simulink model "TractorTransmissionTradeOff"  (R2025a)
settings: Solver=daessc  StartTime=0.0  StopTime=125  RelTol=1e-3  AbsTol=1e-3
PreLoadFcn:
  | distanceVector = [0,0.1389,0.4167,0.8333,1.3889,2.0833,2.9167,3.889,5,6.25,7.6389,200];
  | targetVelocityVector = [0,0.5,1,1.5,2,2.5,3,3.5,4,4.5,5,5];
InitFcn:
  | TractorEnergyComputationInput
undefined symbols (not defined in the file or in its folder): engine, implement, tc, tire, tk, tphi, tykc, tykphi, tyn
libraries: nesl_utility x33, fl_lib x18, sdl_lib x6, simulink x5, slpidlib x1
(part 1 of 3)
CloseFcn:
  | try,close(hTractorTransmissionTradeOff),end
  | clear hTractorTransmissionTradeOff
  | 
  | clear tout simlogTractorTransmissionTradeOff
  | clear logsoutTractorTransmissionTradeOff
  | 
  | clear driveline engine finalDrive
  | clear hydrostaticCVT pump tire implement
  | clear h1_plotEnergySankey
Description:
  | Tractor Transmission Energy Flow Chart
settings Model: Creator=The MathWorks, Inc.  LastModifiedBy=varora
settings SolverCC: AutoScaleAbsTol=off  MaxConsecutiveMinStep=10  AlgebraicLoopSolver=TrustRegion  MaxZcPerStep=1.0
settings DataIOCC: DSMLogging=off  ReturnWorkspaceOutputs=off  SignalLoggingName=logsoutTractorTransmissionTradeOff
settings OptimizationCC: ReuseModelBlockBuffer=off
settings DebuggingCC: IgnoredZcDiagnostic=none  UnconnectedInputMsg=warning  UnconnectedOutputMsg=warning  UnconnectedLineMsg=warning  SymbolicDimsDataTypeCodeGenerationDiagnostic=none
settings ModelReferenceCC: EnableRefExpFcnMdlSchedulingChecks=on
settings SFSimCC: CustomCodeUndefinedFunction=UseInterfaceOnly
settings RTWCC: GPUComputeCapability=3.5  DLArmComputeVersion=19.05
settings SimscapeCC: SimscapeLogName=simlogTractorTransmissionTradeOff  SimscapeLogDataHistory=1000000.0

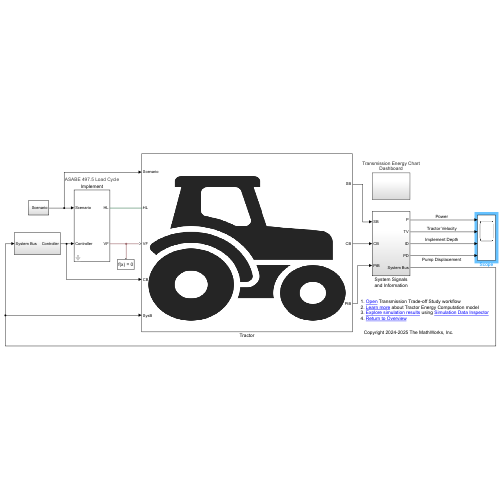
[thumbnail: Simulink's stored preview of the top-level diagram]
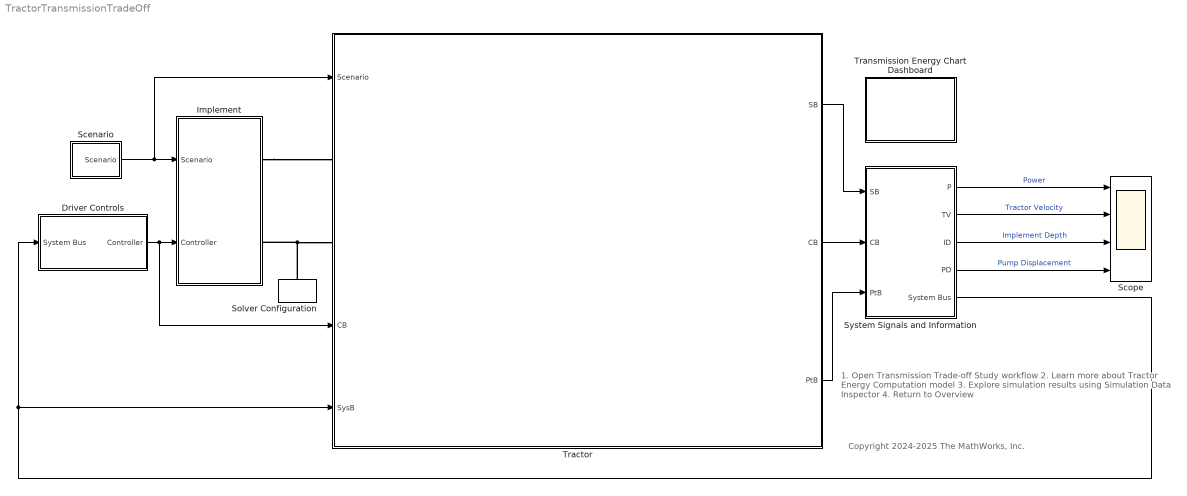
== system TractorTransmissionTradeOff ==
  note: Copyright 2024-2025 The MathWorks, Inc.
  note: 1. Open Transmission Trade-off Study workflow
      | 2. Learn more about Tractor Energy Computation model
      | 3. Explore simulation results using Simulation Data Inspector
      | 4. Return to Overview
  Driver Controls : Subsystem
  Implement : Subsystem  Tag=ASABE 497.5 Load Cycle  Description=ASABE 497.5 Load Cycle  mask{methodForceComputation=Draft force prediction based on ASABE D497.5 standard, typeImplement=Chisel Plow - 5 cm straight point, widthImplement=1, numberTools=implement.numberTools, angleRake=implement.angleRake, vectorVelocity=[-1,0,0.05,0.5,1,1.5], vectorDraft=[-2.5,0,1800,2260,2480,2700], vectorVF=[0.5,0,-480,-525,-580,-620]}
      mask prompts: methodForceComputation "Draft (horizontal) force and vertical force computation"; typeImplement "Implement type"; widthImplement "Implement width (m)"; numberTools "Number of tools"; angleRake "Implement rake angle (deg)"; vectorVelocity "Velocity vector (m/s)"; vectorDraft "Draft force vector (N)"; vectorVF "Vertical force vector (N)"
      settings: AttributesFormatString=%<Tag>
      mask Callback methodForceComputation: ImplementMask
      mask Callback typeImplement: ImplementMask
      mask Callback widthImplement: ImplementMask
      mask Callback numberTools: ImplementMask
      mask Callback angleRake: ImplementMask
      mask Callback vectorVelocity: ImplementMask
      mask Callback vectorDraft: ImplementMask
      mask Callback vectorVF: ImplementMask
  Scenario : Subsystem
      settings: PortSchema="{\"entries\":[{\"content\":{\"sides\":[{\"content\":{\"connectorIds\":[\"Out1\"]},\"type\":\"ConnectorPlacement.EquallySpacedRectSide\",\"uuid\":\"b29e7b9e-789a-4413-ae11-5995fbedc15e\"},{\"content\":{\"side\":\"RIGHT\"},\"type\":\"ConnectorPlacement.EquallySpacedRectSide\",\"uuid\":\"46779515-8d36-4954-9a1a-0bbe9b69e0ab\"},{\"content\":{\"side\":\"TOP\"},\"type\":\"ConnectorPlacement.EquallySpacedRectSide\",\"uuid\":\"af37b6bf-e8aa-4a9f-b639-d899b0359ee5\"}]},\"type\":\"ConnectorPlacement.EquallySpacedConnector\",\"uuid\":\"f01fcd35-a429-4c8a-8cd6-eccdc9914f9f\"}],\"packageUris\":[\"http://schema.mathworks.com/mf0/Connector/R2020b\"],\"version\":\"1.0\"}"
  Scope : Scope  NumInputPorts=4
      settings: Title=Power, CVT (kW)  ActiveDisplayYMinimum=-3.21446  ActiveDisplayYMaximum=28.93014
  Solver Configuration : nesl_utility/Solver Configuration  PhysicalDomain=network_engine_domain  SubClassName=solver  LeftPortType=input  RightPortType=generic  Tones=[]  Harmonics=[]  SimulateNoise=off  Profile=off  UseLocalSampling=off  EnableSwitchedLinearOptims=on  FrequencyDomain=off  UseCCode=off  RelTol=0.001  AbsTol=1e-06  MinStep=1e-09  ToWorkspace=off  RevertToSquareIcSolve=off  NumHomotopyIterations=100  PhasorMode=off  PhasorModeNumHarmonics=1  ConsistencySolver=NEWTON_FTOL  IndexReductionMethod=DerivativeReplacement  DoDC=off  ResidualTolerance=1e-09  ConsistencyTolSource=GLOBAL  ConsistencyAbsTol=0.001  ConsistencyRelTol=0.001  ConsistencyTolFactor=0.001  UseLocalSolver=off  LocalSolverChoice=NE_BACKWARD_EULER_ADVANCER  ResolveIndetEquations=on  FunctionEvalNumThread=1  LocalSolverSampleTime=1e-5  DoFixedCost=off  MaxNonlinIter=6  MaxModeIter=2  ComputeImpulses=off  ImpulseIterations=2  LinearAlgebra=auto  LinearAlgebraNumThread=0  EquationFormulation=NE_TIME_EF  DelaysMemoryBudget=1024  AutomaticFiltering=on  FilteringTimeConstant=0.001  PartitionStorageMethod=AS_NEEDED  PartitionMemoryBudget=1024  PartitionMethod=ROBUST  MultibodyUseLocalSolver=off  MultibodyLocalSolverChoice=ODE1  MultibodyLocalSolverSampleTime=0.001
  System Signals and Information : Subsystem
  Tractor : Subsystem
      settings: PortSchema="{\"entries\":[{\"content\":{\"sides\":[{\"content\":{\"connectorIds\":[\"In1\",\"LConn1\",\"LConn2\",\"In2\",\"In3\"]},\"type\":\"ConnectorPlacement.EquallySpacedRectSide\",\"uuid\":\"54713dc4-af1f-4753-ac81-fb7b321017cb\"},{\"content\":{\"connectorIds\":[\"Out1\",\"Out2\",\"Out3\"],\"side\":\"RIGHT\"},\"type\":\"ConnectorPlacement.EquallySpacedRectSide\",\"uuid\":\"1649f1ef-bc57-4766-b2b0-80ad557aa9be\"},{\"content\":{\"side\":\"TOP\"},\"type\":\"ConnectorPlacement.EquallySpacedRectSide\",\"uuid\":\"7ab6efae-1587-4e38-886b-370438e4a6fb\"}]},\"type\":\"ConnectorPlacement.EquallySpacedConnector\",\"uuid\":\"47a9668e-68aa-4ab4-a25a-cd113bc06b02\"}],\"packageUris\":[\"http://schema.mathworks.com/mf0/Connector/R2020b\"],\"version\":\"1.0\"}"
      mask Display: image('FullTractor.png');
  Transmission Energy Chart Dashboard : Subsystem
  wires:
  System Signals and Information/3(ID) -> Scope/3  "Implement Depth"
  System Signals and Information/2(TV) -> Scope/2  "Tractor Velocity"
  System Signals and Information/1(P) -> Scope/1  "Power"
  Tractor/3(PtB) -> System Signals and Information/3(PtB)
  Tractor/1(SB) -> System Signals and Information/1(SB)
  Scenario/1(Scenario) -> Tractor/1(Scenario), Implement/1(Scenario)
  Driver Controls/1(Controller) -> Tractor/2("CB "), Implement/2(Controller)
  Tractor/2(CB) -> System Signals and Information/2(CB)
  System Signals and Information/4(PD) -> Scope/4  "Pump Displacement"
  System Signals and Information/5(System Bus) -> Tractor/3(SysB), Driver Controls/1(System Bus)
  connections:
  Implement/RConn1 -- Tractor/LConn1
  Solver Configuration/RConn1 -- Implement/RConn2 -- Tractor/LConn2

== system TractorTransmissionTradeOff/Driver Controls ==
  System Bus : Inport
  Bus Selector : BusSelector  OutputSignals=Tractor Velocity
  CVT Control System : Subsystem
  Engine Speed Command : Subsystem
  Implement Depth Command : Subsystem
  Bus Element Out : Outport  PortName=Controller  Element=Implement Depth Command
  Bus Element Out1 : Outport  PortName=Controller  Element=Speed Command
  Bus Element Out2 : Outport  PortName=Controller  Element=Pump Displacement
  wires:
  Implement Depth Command/1(Depth Command) -> Bus Element Out/1
  CVT Control System/1(Pump Displacement) -> Bus Element Out2/1
  System Bus/1 -> Bus Selector/1
  Bus Selector/1 -> CVT Control System/1(Tractor Vel)  "<Tractor Velocity>"
  Engine Speed Command/1(Engine Speed) -> Bus Element Out1/1

== system TractorTransmissionTradeOff/Implement ==
  note: Implement connectivity
  note: Connectivity bet ween Implement block and bus signals from Scenario and Controller are enabled or disabled based on the dropdown option for 'Draft (horizontal) force and vertical force computation' parameter in the Implement masked subsystem. This is achieved by enabling/ disabling the following:
      |
      | 1. Line connectivity from Simulink-PS Converter & Simulink-PS Converter1 blocks to Implement block.
      | 2. Simulink-PS Converter & Simulink-PS Converter1 blocks (commenting on/ off)
      | 3. Line connectivity from Bus Selector and Bus Selector1 to Terminators subsystem.
      | 4. Terminators subsystem (commenting on/ off).
  Scenario : Inport
  Controller : Inport  Port=2
  Bus Selector : BusSelector  OutputSignals=Implement-Soil Parameter
  Bus Selector1 : BusSelector  OutputSignals=Implement Depth Command
  Implement : SimscapeComponentBlock  SourceFile=implement  ComponentPath=implement  ComponentVariants="[\"implement\"]"  ComponentVariantNames="[\"implement\"]"  ClassName=implement  SchemaVersion=1  parameterization=ForceComputation.Calculate  type_implement=ImplementType.ChiselPlow  width_implement=1 m  number_tools=5  rake_angle=55 deg  velocity_vector=[-1 0 0.05 0.5 1 1.5] m/s  draft_vector=[-2.5 0 1800 2260 2480 2700] N  VF_vector=[0.5 0 -480 -525 -580 -620] N  velocity_thr=0.001 m/s  depth_min=0.01 cm
      settings: CopyFcn=simscape.sscblock.internal.componentBlockCallback(gcbh,'COPY')  PreCopyFcn=simscape.sscblock.internal.componentBlockCallback(gcbh,'PRECOPY')  PreDeleteFcn=simscape.sscblock.internal.componentBlockCallback(gcbh,'PREDELETE')  InternalSimscapePortConfiguration="{\"Bottom\":[{\"id\":\"VF\",\"label\":\"VF\",\"type\":\"output\"}],\"Left\":[{\"id\":\"texture_soil_input\",\"label\":\"ST\",\"type\":\"input\"},{\"id\":\"depth_tillage\",\"label\":\"d\",\"type\":\"input\"}],\"Right\":[{\"id\":\"H\",\"label\":\"H\",\"type\":\"foundation.mechanical.translational.translational\"}],\"Top\":[]}"
      mask Type: Implement
  Simulink-PS Converter1 : nesl_utility/Simulink-PS Converter  PhysicalDomain=network_engine_domain  SubClassName=ps_input  LeftPortType=input  RightPortType=output  PseudoPeriodic=off  Frequencies=[]  NoiseDistribution=none  NoiseParameters=[]  Unit=cm  AffineConversion=off  FilteringAndDerivatives=provide  SimscapeFilterOrder=1  InputFilterTimeConstant=0.001  UdotUserProvided=0
  Simulink-PS Converter : nesl_utility/Simulink-PS Converter  PhysicalDomain=network_engine_domain  SubClassName=ps_input  LeftPortType=input  RightPortType=output  PseudoPeriodic=off  Frequencies=[]  NoiseDistribution=none  NoiseParameters=[]  Unit=1  AffineConversion=off  FilteringAndDerivatives=provide  SimscapeFilterOrder=1  InputFilterTimeConstant=0.001  UdotUserProvided=0
  Terminators : Subsystem  Commented=on
      mask Display: disp('T')
  HL : PMIOPort  Side=Right
  VF : PMIOPort  Port=2  Side=Right
  wires:
  Scenario/1 -> Bus Selector/1
  Bus Selector/1 -> Simulink-PS Converter/1  "<Implement-Soil Parameter>"
  Controller/1 -> Bus Selector1/1
  Bus Selector1/1 -> Simulink-PS Converter1/1  "<Implement Depth Command>"
  connections:
  HL/RConn1 -- Implement/RConn1
  VF/RConn1 -- Implement/RConn2
  Simulink-PS Converter/RConn1 -- Implement/LConn1
  Simulink-PS Converter1/RConn1 -- Implement/LConn2

== system TractorTransmissionTradeOff/Scenario ==
  note: Scenario subsystem description
  note: You can define terrain properties and tire-soil interaction
      | properties in the <> tire parameters subsystem.
      | You can define soil texture in the Implement-Soil Scenario subsystem.
      | You can define road inclination in the Road Inclination Scenario subsystem.
  Front Left Tire Parameters : Subsystem
  Front Right Tire Parameters : Subsystem
  Implement-Soil Scenario : Subsystem  mask{textureSoil=Coarse}
      mask prompts: textureSoil "Soil texture"
      mask init:
      | switch textureSoil
      |     case 'Fine'
      |         textureID = 1;
      |     case 'Medium'
      |         textureID = 2;
      |     case 'Coarse'
      |         textureID = 3;
      | end
  Rear Right Tire Parameters : Subsystem
  RearLeft Tire Parameters : Subsystem
  Road Inclination Scenario : Subsystem
  Bus Element Out : Outport  PortName=Scenario  Element=Front Left Tire
  Bus Element Out1 : Outport  PortName=Scenario  Element=Front Right Tire
  Bus Element Out2 : Outport  PortName=Scenario  Element=Rear Left Tire
  Bus Element Out3 : Outport  PortName=Scenario  Element=Rear Right Tire
  Bus Element Out4 : Outport  PortName=Scenario  Element=Implement-Soil Parameter
  BusElementOut : Outport  PortName=Scenario  Element=Road Inclination
  wires:
  Front Left Tire Parameters/1(Front Left Tire Bus) -> Bus Element Out/1
  Front Right Tire Parameters/1(Front Right Tire Bus) -> Bus Element Out1/1
  Rear Right Tire Parameters/1(Rear Right Tire Bus) -> Bus Element Out3/1
  RearLeft Tire Parameters/1(Rear Left Tire Bus) -> Bus Element Out2/1
  Implement-Soil Scenario/1(Implement-Soil Parameter) -> Bus Element Out4/1
  Road Inclination Scenario/1(Scenario) -> BusElementOut/1

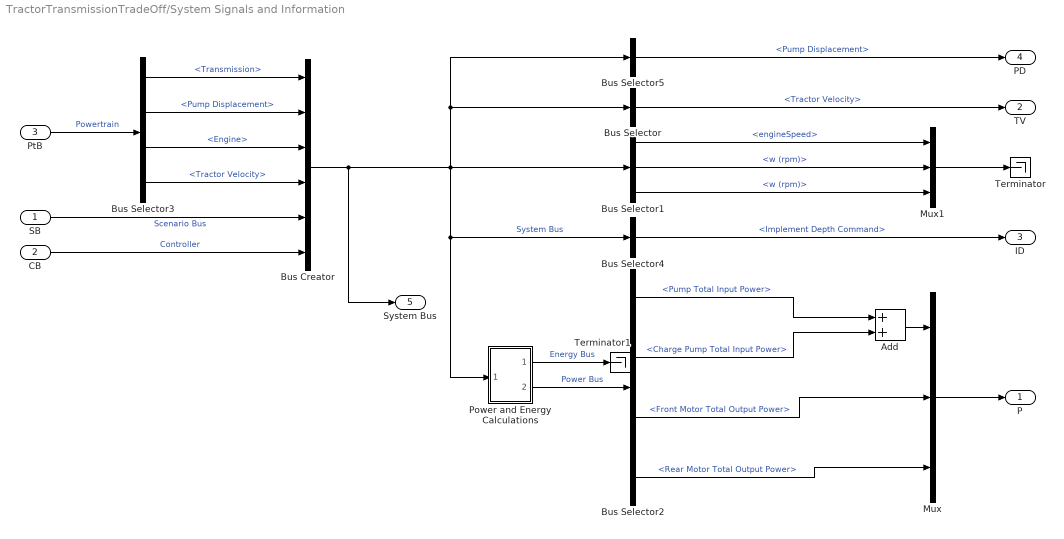
== system TractorTransmissionTradeOff/System Signals and Information ==
  SB : Inport
  CB : Inport  Port=2
  PtB : Inport  Port=3
  Add : Sum
  Bus Creator : BusCreator  Inputs=6
  Bus Selector : BusSelector  OutputSignals=Tractor Velocity
  Bus Selector1 : BusSelector  OutputSignals=Engine.engineSpeed,Transmission.Front Motor.w (rpm),Transmission.Rear Motor.w (rpm)
  Bus Selector2 : BusSelector  OutputSignals=Pump Total Input Power,Charge Pump Total Input Power,Front Motor Total Output Power,Rear Motor Total Output Power
  Bus Selector3 : BusSelector  OutputSignals=Transmission,Pump Displacement,Engine,Tractor Velocity
  Bus Selector4 : BusSelector  OutputSignals=Controller.Implement Depth Command
  Bus Selector5 : BusSelector  OutputSignals=Pump Displacement
  Mux : Mux  Inputs=3
  Mux1 : Mux  Inputs=3
  Power and Energy Calculations : Subsystem
      mask Display: image('Energy.png'); % Use "Edit Image" on toolstrip to change.
  Terminator : Terminator
  Terminator1 : Terminator
  P : Outport
  TV : Outport  Port=2
  ID : Outport  Port=3
  PD : Outport  Port=4
  System Bus : Outport  Port=5
  wires:
  Mux/1 -> P/1
  Bus Selector3/1 -> Bus Creator/1  "<Transmission>"
  Bus Selector3/2 -> Bus Creator/2  "<Pump Displacement>"
  Bus Selector3/3 -> Bus Creator/3  "<Engine>"
  Bus Selector3/4 -> Bus Creator/4  "<Tractor Velocity>"
  Bus Creator/1 -> System Bus/1, Bus Selector1/1, Bus Selector5/1, Bus Selector/1, Power and Energy Calculations/1(System Bus), Bus Selector4/1  "System Bus"
  Bus Selector1/1 -> Mux1/1  "<engineSpeed>"
  Bus Selector1/3 -> Mux1/3  "<w (rpm)>"
  PtB/1 -> Bus Selector3/1  "Powertrain"
  Bus Selector/1 -> TV/1  "<Tractor Velocity>"
  SB/1 -> Bus Creator/5  "Scenario Bus"
  CB/1 -> Bus Creator/6  "Controller"
  Power and Energy Calculations/1(Energy Bus) -> Terminator1/1  "Energy Bus"
  Bus Selector1/2 -> Mux1/2  "<w (rpm)>"
  Bus Selector4/1 -> ID/1  "<Implement Depth Command>"
  Mux1/1 -> Terminator/1
  Bus Selector2/1 -> Add/1  "<Pump Total Input Power>"
  Bus Selector2/2 -> Add/2  "<Charge Pump Total Input Power>"
  Add/1 -> Mux/1
  Power and Energy Calculations/2(Power Bus) -> Bus Selector2/1  "Power Bus"
  Bus Selector2/3 -> Mux/2  "<Front Motor Total Output Power>"
  Bus Selector2/4 -> Mux/3  "<Rear Motor Total Output Power>"
  Bus Selector5/1 -> PD/1  "<Pump Displacement>"

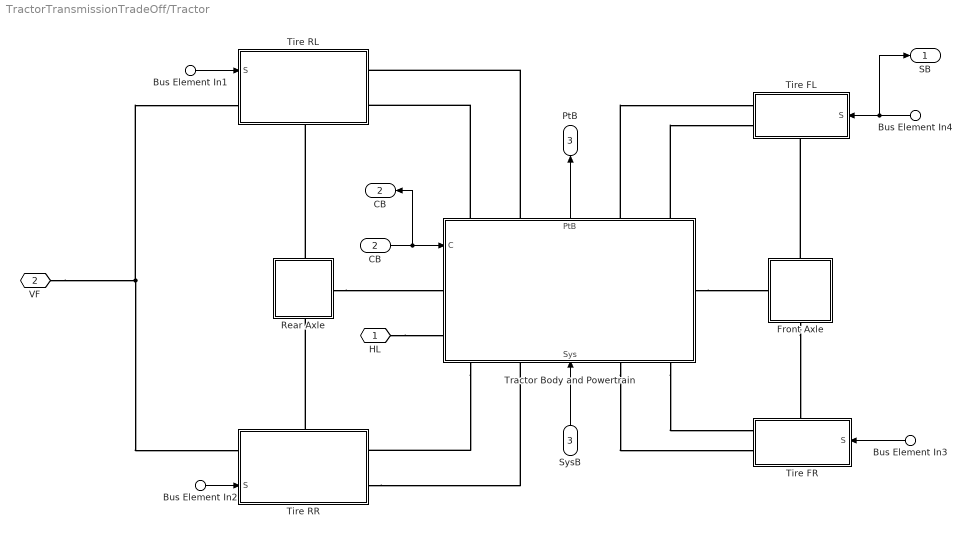
== system TractorTransmissionTradeOff/Tractor ==
  Bus Element In{1..4} (4 alike) : Inport  PortName=Scenario
  "CB " : Inport  Port=2
  SysB : Inport  Port=3
  Front Axle : Subsystem
      settings: PortSchema="{\"entries\":[{\"content\":{\"sides\":[{\"content\":{},\"type\":\"ConnectorPlacement.EquallySpacedRectSide\",\"uuid\":\"026b5002-63df-4b45-94ce-e3e456531417\"},{\"content\":{\"connectorIds\":[\"RConn1\"],\"side\":\"RIGHT\"},\"type\":\"ConnectorPlacement.EquallySpacedRectSide\",\"uuid\":\"9a3773c6-ea4f-4541-b847-4aeb1357eea4\"},{\"content\":{\"connectorIds\":[\"LConn1\"],\"side\":\"TOP\"},\"type\":\"ConnectorPlacement.EquallySpacedRectSide\",\"uuid\":\"09b6a560-9219-4e81-a680-51bb22d5804b\"},{\"content\":{\"connectorIds\":[\"RConn2\"],\"side\":\"BOTTOM\"},\"type\":\"ConnectorPlacement.EquallySpacedRectSide\",\"uuid\":\"b003a922-06ca-4cc0-b2d6-10676bcbd4b4\"}]},\"type\":\"ConnectorPlacement.EquallySpacedConnector\",\"uuid\":\"e2257446-62b4-4aca-ac75-a234c474d310\"}],\"packageUris\":[\"http://schema.mathworks.com/mf0/Connector/R2020b\"],\"version\":\"1.0\"}"
  Rear Axle : Subsystem
      settings: PortSchema="{\"entries\":[{\"content\":{\"sides\":[{\"content\":{},\"type\":\"ConnectorPlacement.EquallySpacedRectSide\",\"uuid\":\"026b5002-63df-4b45-94ce-e3e456531417\"},{\"content\":{\"connectorIds\":[\"RConn1\"],\"side\":\"RIGHT\"},\"type\":\"ConnectorPlacement.EquallySpacedRectSide\",\"uuid\":\"9a3773c6-ea4f-4541-b847-4aeb1357eea4\"},{\"content\":{\"connectorIds\":[\"LConn1\"],\"side\":\"TOP\"},\"type\":\"ConnectorPlacement.EquallySpacedRectSide\",\"uuid\":\"09b6a560-9219-4e81-a680-51bb22d5804b\"},{\"content\":{\"connectorIds\":[\"RConn2\"],\"side\":\"BOTTOM\"},\"type\":\"ConnectorPlacement.EquallySpacedRectSide\",\"uuid\":\"5183298d-70d1-4b83-bb90-8882b3619986\"}]},\"type\":\"ConnectorPlacement.EquallySpacedConnector\",\"uuid\":\"e2257446-62b4-4aca-ac75-a234c474d310\"}],\"packageUris\":[\"http://schema.mathworks.com/mf0/Connector/R2020b\"],\"version\":\"1.0\"}"
  Tire FL : Subsystem
      settings: PortSchema="{\"entries\":[{\"content\":{\"sides\":[{\"content\":{\"connectorIds\":[\"LConn1\",\"LConn2\"]},\"type\":\"ConnectorPlacement.EquallySpacedRectSide\",\"uuid\":\"0e9833ab-dd86-46ea-ab64-a65b439bce81\"},{\"content\":{\"connectorIds\":[\"In1\"],\"side\":\"RIGHT\"},\"type\":\"ConnectorPlacement.EquallySpacedRectSide\",\"uuid\":\"36c5dd6e-c752-4ac3-a0c1-2f37b7fd136a\"},{\"content\":{\"side\":\"TOP\"},\"type\":\"ConnectorPlacement.EquallySpacedRectSide\",\"uuid\":\"0bd2a76b-741b-400c-a193-5ed7d3d369d2\"},{\"content\":{\"connectorIds\":[\"RConn1\"],\"side\":\"BOTTOM\"},\"type\":\"ConnectorPlacement.EquallySpacedRectSide\",\"uuid\":\"8a0bdfa8-eaf0-4519-ae75-c3bcc22df53a\"}]},\"type\":\"ConnectorPlacement.EquallySpacedConnector\",\"uuid\":\"5906df78-5ca5-40a2-9fe4-964fd15007ab\"}],\"packageUris\":[\"http://schema.mathworks.com/mf0/Connector/R2020b\"],\"version\":\"1.0\"}"
  Tire FR : Subsystem
      settings: PortSchema="{\"entries\":[{\"content\":{\"sides\":[{\"content\":{\"connectorIds\":[\"LConn1\",\"LConn2\"]},\"type\":\"ConnectorPlacement.EquallySpacedRectSide\",\"uuid\":\"7d1ae1e2-2517-4b59-9e4a-0cb77dd3afd7\"},{\"content\":{\"connectorIds\":[\"In1\"],\"side\":\"RIGHT\"},\"type\":\"ConnectorPlacement.EquallySpacedRectSide\",\"uuid\":\"11157514-b90b-4d82-9f7b-3cd850b5f5ac\"},{\"content\":{\"connectorIds\":[\"LConn3\"],\"side\":\"TOP\"},\"type\":\"ConnectorPlacement.EquallySpacedRectSide\",\"uuid\":\"4d99c937-f663-4199-8015-5fa41e849046\"}]},\"type\":\"ConnectorPlacement.EquallySpacedConnector\",\"uuid\":\"3f82b3de-dae1-4ac7-bdf5-b82b10b3e59d\"}],\"packageUris\":[\"http://schema.mathworks.com/mf0/Connector/R2020b\"],\"version\":\"1.0\"}"
  Tire RL : Subsystem
      settings: PortSchema="{\"entries\":[{\"content\":{\"sides\":[{\"content\":{\"connectorIds\":[\"LConn1\",\"LConn2\"]},\"type\":\"ConnectorPlacement.EquallySpacedRectSide\",\"uuid\":\"1448c855-24f3-49ae-9934-34df724fc47f\"},{\"content\":{\"connectorIds\":[\"In1\",\"RConn1\"],\"side\":\"RIGHT\"},\"type\":\"ConnectorPlacement.EquallySpacedRectSide\",\"uuid\":\"df2e3118-cf50-4ee3-834c-d668683399be\"},{\"content\":{\"side\":\"TOP\"},\"type\":\"ConnectorPlacement.EquallySpacedRectSide\",\"uuid\":\"4a478f8a-f8bb-4588-bb4c-2f0b807fe55a\"},{\"content\":{\"connectorIds\":[\"RConn2\"],\"side\":\"BOTTOM\"},\"type\":\"ConnectorPlacement.EquallySpacedRectSide\",\"uuid\":\"80dd0032-136d-4f5c-8cee-4346ded75175\"}]},\"type\":\"ConnectorPlacement.EquallySpacedConnector\",\"uuid\":\"fd19bf53-ddb4-4ab6-b0a8-e39c218bcbd7\"}],\"packageUris\":[\"http://schema.mathworks.com/mf0/Connector/R2020b\"],\"version\":\"1.0\"}"
  Tire RR : Subsystem
      settings: PortSchema="{\"entries\":[{\"content\":{\"sides\":[{\"content\":{\"connectorIds\":[\"LConn1\",\"LConn2\"]},\"type\":\"ConnectorPlacement.EquallySpacedRectSide\",\"uuid\":\"7d1ae1e2-2517-4b59-9e4a-0cb77dd3afd7\"},{\"content\":{\"connectorIds\":[\"RConn1\",\"In1\"],\"side\":\"RIGHT\"},\"type\":\"ConnectorPlacement.EquallySpacedRectSide\",\"uuid\":\"11157514-b90b-4d82-9f7b-3cd850b5f5ac\"},{\"content\":{\"connectorIds\":[\"LConn3\"],\"side\":\"TOP\"},\"type\":\"ConnectorPlacement.EquallySpacedRectSide\",\"uuid\":\"4d99c937-f663-4199-8015-5fa41e849046\"}]},\"type\":\"ConnectorPlacement.EquallySpacedConnector\",\"uuid\":\"3f82b3de-dae1-4ac7-bdf5-b82b10b3e59d\"}],\"packageUris\":[\"http://schema.mathworks.com/mf0/Connector/R2020b\"],\"version\":\"1.0\"}"
  Tractor Body and Powertrain : Subsystem
      settings: PortSchema="{\"entries\":[{\"content\":{\"sides\":[{\"content\":{\"connectorIds\":[\"In1\",\"LConn1\",\"LConn2\"]},\"type\":\"ConnectorPlacement.EquallySpacedRectSide\",\"uuid\":\"05c05ec9-2fff-417f-bd83-012fb1f38f87\"},{\"content\":{\"connectorIds\":[\"RConn1\"],\"side\":\"RIGHT\"},\"type\":\"ConnectorPlacement.EquallySpacedRectSide\",\"uuid\":\"aa1d2bbf-9e9a-488d-bbfb-b2324626d545\"},{\"content\":{\"connectorIds\":[\"LConn3\",\"LConn4\",\"Out1\",\"LConn5\",\"LConn6\"],\"side\":\"TOP\"},\"type\":\"ConnectorPlacement.EquallySpacedRectSide\",\"uuid\":\"c7d7f598-6e33-4c01-b25f-48e4a93da769\"},{\"content\":{\"connectorIds\":[\"RConn2\",\"RConn3\",\"In2\",\"RConn4\",\"RConn5\"],\"side\":\"BOTTOM\"},\"type\":\"ConnectorPlacement.EquallySpacedRectSide\",\"uuid\":\"9bed1270-7dff-472f-a56d-a46898bffafb\"}]},\"type\":\"ConnectorPlacement.EquallySpacedConnector\",\"uuid\":\"705bb31f-0b66-4068-8292-9833bb38fc86\"}],\"packageUris\":[\"http://schema.mathworks.com/mf0/Connector/R2020b\"],\"version\":\"1.0\"}"
      mask Display: disp('Tractor Body and Powertrain');
  HL : PMIOPort  Side=Left
  VF : PMIOPort  Port=2  Side=Left
  SB : Outport
  CB : Outport  Port=2
  PtB : Outport  Port=3
  wires:
  Tractor Body and Powertrain/1(PtB) -> PtB/1
  Bus Element In2/1 -> Tire RR/1(S)
  Bus Element In4/1 -> Tire FL/1(S), SB/1
  Bus Element In1/1 -> Tire RL/1(S)
  Bus Element In3/1 -> Tire FR/1(S)
  "CB "/1 -> CB/1, Tractor Body and Powertrain/1(C)
  SysB/1 -> Tractor Body and Powertrain/2(Sys)
  connections:
  Tractor Body and Powertrain/LConn5 -- Tire FL/LConn1
  Tractor Body and Powertrain/LConn6 -- Tire FL/LConn2
  Tractor Body and Powertrain/LConn3 -- Tire RL/LConn2
  Tire RR/LConn2 -- Tractor Body and Powertrain/RConn3
  Tractor Body and Powertrain/LConn4 -- Tire RL/LConn1
  Tractor Body and Powertrain/RConn4 -- Tire FR/LConn2
  Tire RR/LConn3 -- Rear Axle/RConn2
  Rear Axle/LConn1 -- Tire RL/RConn2
  Front Axle/RConn2 -- Tire FR/LConn3
  Tractor Body and Powertrain/RConn2 -- Tire RR/LConn1
  Tractor Body and Powertrain/RConn5 -- Tire FR/LConn1
  Front Axle/LConn1 -- Tire FL/RConn1
  HL/RConn1 -- Tractor Body and Powertrain/LConn2
  Tractor Body and Powertrain/RConn1 -- Front Axle/RConn1
  Rear Axle/RConn1 -- Tractor Body and Powertrain/LConn1
  VF/RConn1 -- Tire RL/RConn1 -- Tire RR/RConn1

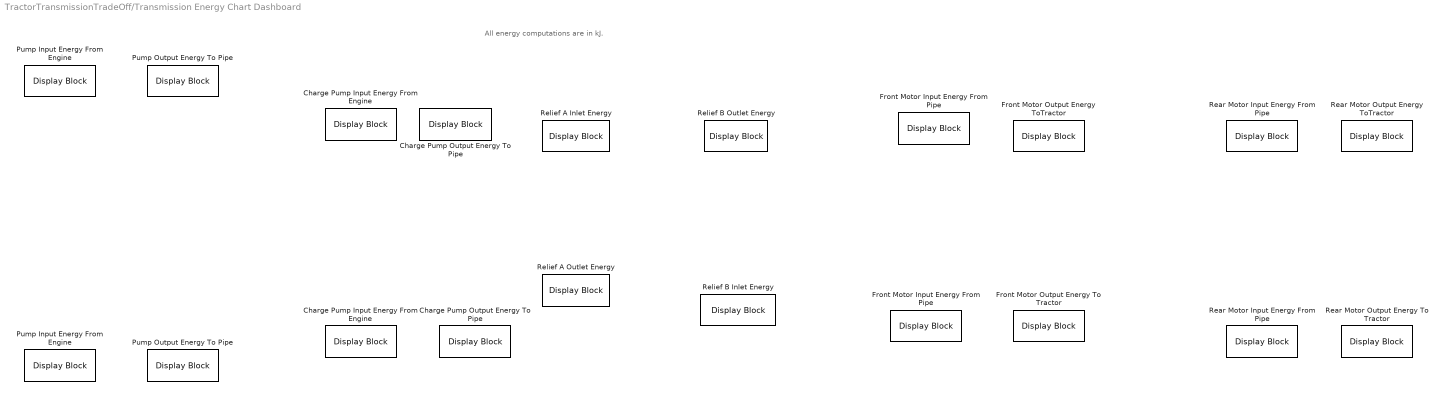
== system TractorTransmissionTradeOff/Transmission Energy Chart Dashboard ==
  note: All energy computations are in kJ.
  Charge Pump Input Energy From Engine : DisplayBlock  LabelPosition=Hide  Format=Integer  Transparency=1  GridColor=[0.502, 0.502, 0.502]
  "Charge Pump Input Energy From Engine " : DisplayBlock  LabelPosition=Hide  Format=Integer  Transparency=1  GridColor=[0.502, 0.502, 0.502]
  Charge Pump Output Energy To Pipe : DisplayBlock  LabelPosition=Hide  Format=Integer  Transparency=1  GridColor=[0.502, 0.502, 0.502]
  "Charge Pump Output Energy To Pipe " : DisplayBlock  LabelPosition=Hide  Format=Integer  Transparency=1  GridColor=[0.502, 0.502, 0.502]
  "Front Motor Output Energy ToTractor " : DisplayBlock  LabelPosition=Hide  Format=Integer  Transparency=1  GridColor=[0.502, 0.502, 0.502]
  Front Motor Output Energy To Tractor : DisplayBlock  LabelPosition=Hide  Format=Integer  Transparency=1  GridColor=[0.502, 0.502, 0.502]
  Front Motor Input Energy From Pipe : DisplayBlock  LabelPosition=Hide  Format=Integer  Transparency=1  GridColor=[0.502, 0.502, 0.502]
  "Front Motor Input Energy From Pipe " : DisplayBlock  LabelPosition=Hide  Format=Integer  Transparency=1  GridColor=[0.502, 0.502, 0.502]
  Pump Input Energy From Engine : DisplayBlock  LabelPosition=Hide  Format=Integer  Transparency=1  GridColor=[0.502, 0.502, 0.502]
  "Pump Input Energy From Engine " : DisplayBlock  LabelPosition=Hide  Format=Integer  Transparency=1  GridColor=[0.502, 0.502, 0.502]
  Pump Output Energy To Pipe : DisplayBlock  LabelPosition=Hide  Format=Integer  Transparency=1  GridColor=[0.502, 0.502, 0.502]
  "Pump Output Energy To Pipe " : DisplayBlock  LabelPosition=Hide  Format=Integer  Transparency=1  GridColor=[0.502, 0.502, 0.502]
  "Rear Motor Output Energy ToTractor " : DisplayBlock  LabelPosition=Hide  Format=Integer  Transparency=1  GridColor=[0.502, 0.502, 0.502]
  Rear Motor Output Energy To Tractor : DisplayBlock  LabelPosition=Hide  Format=Integer  Transparency=1  GridColor=[0.502, 0.502, 0.502]
  Rear Motor Input Energy From Pipe : DisplayBlock  LabelPosition=Hide  Format=Integer  Transparency=1  GridColor=[0.502, 0.502, 0.502]
  "Rear Motor Input Energy From Pipe " : DisplayBlock  LabelPosition=Hide  Format=Integer  Transparency=1  GridColor=[0.502, 0.502, 0.502]
  Relief A Inlet Energy : DisplayBlock  LabelPosition=Hide  Format=Integer  Transparency=1  GridColor=[0.502, 0.502, 0.502]
  Relief A Outlet Energy : DisplayBlock  LabelPosition=Hide  Format=Integer  Transparency=1  GridColor=[0.502, 0.502, 0.502]
  Relief B Inlet Energy : DisplayBlock  LabelPosition=Hide  Format=Integer  Transparency=1  GridColor=[0.502, 0.502, 0.502]
  Relief B Outlet Energy : DisplayBlock  LabelPosition=Hide  Format=Integer  Transparency=1  GridColor=[0.502, 0.502, 0.502]

== system TractorTransmissionTradeOff/Driver Controls/CVT Control System ==
  Tractor Vel : Inport
  PID Controller : slpidlib/PID Controller  Controller=PID  Form=Parallel  TimeDomain=Continuous-time  UseExternalTs=off  SampleTime=-1  IntegratorMethod=Forward Euler  FilterMethod=Forward Euler  ControllerParametersSource=internal  P=75  I=10  UseKiTs=off  D=0  UseExternalDerivativeSource=off  N=100  UseFilter=on  TunerSelectOption=Transfer Function Based (PID Tuner App)  InitialConditionSource=internal  InitialConditionForIntegrator=0  InitialConditionForFilter=0  DifferentiatorICPrevScaledInput=0  ExternalReset=none  TrackingMode=off  Kt=1  LimitOutput=off  SatLimitsSource=internal  UpperSaturationLimit=inf  LowerSaturationLimit=-inf  LinearizeAsGain=on  AntiWindupMode=none  Kb=1  LimitIntegrator=off  UpperIntegratorSaturationLimit=inf  LowerIntegratorSaturationLimit=-inf  POutMin=[]  POutMax=[]  IOutMin=[]  IOutMax=[]  DOutMin=[]  DOutMax=[]  NOutMin=[]  NOutMax=[]  SumOutMin=[]  SumOutMax=[]  SaturationOutMin=[]  SaturationOutMax=[]  PParamMin=[]  PParamMax=[]  IParamMin=[]  IParamMax=[]  DParamMin=[]  DParamMax=[]  NParamMin=[]  NParamMax=[]  KbParamMin=[]  KbParamMax=[]  KtParamMin=[]  KtParamMax=[]  KbOutMin=[]  KbOutMax=[]  KtOutMin=[]  KtOutMax=[]  IntegratorOutMin=[]  IntegratorOutMax=[]  FilterOutMin=[]  FilterOutMax=[]  SumI1OutMin=[]  SumI1OutMax=[]  SumI2OutMin=[]  SumI2OutMax=[]  SumI3OutMin=[]  SumI3OutMax=[]  SumI4OutMin=[]  SumI4OutMax=[]  SumDOutMin=[]  SumDOutMax=[]  DifferentiatorOutMin=[]  DifferentiatorOutMax=[]  FilterDiffOutCoefMin=[]  FilterDiffOutCoefMax=[]  ReciprocalOutMin=[]  ReciprocalOutMax=[]  SumDenOutMin=[]  SumDenOutMax=[]  SumNumOutMin=[]  SumNumOutMax=[]  DivideOutMin=[]  DivideOutMax=[]  UdiffTsProdOutMin=[]  UdiffTsProdOutMax=[]  NTsProdOutMin=[]  NTsProdOutMax=[]  UintegralTsProdOutMin=[]  UintegralTsProdOutMax=[]  UngainTsProdOutMin=[]  UngainTsProdOutMax=[]  ClampingZeroOutDataTypeStr=Inherit: Inherit via back propagation  ClampingZeroOutMin=[]  ClampingZeroOutMax=[]  FilterDenConstantOutDataTypeStr=Inherit: Inherit via back propagation  FilterDenConstantOutMin=[]  FilterDenConstantOutMax=[]  PCopyOutDataTypeStr=Inherit: Inherit via back propagation  PCopyOutMin=[]  PCopyOutMax=[]  NCopyOutDataTypeStr=Inherit: Inherit via back propagation  NCopyOutMin=[]  NCopyOutMax=[]  IntegratorContinuousStateAttributes=''  IntegratorStateMustResolveToSignalObject=off  IntegratorRTWStateStorageClass=Auto  FilterContinuousStateAttributes=''  FilterStateMustResolveToSignalObject=off  FilterRTWStateStorageClass=Auto  ParallelPVariant=InternalParameters  IdealPVariant=Disabled  IVariant=InternalParameters  DVariant=InternalParameters  IntegratorVariant=Continuous  SatVariant=Disabled  AWVariant=Passthrough  PCopyVariant=Disabled  TRVariant=Disabled  FdbkBlocksVariant=Forward  IdealPFdbkVariant=Disabled  SatFdbkVariant=Disabled  DerivativeFilterVariant=ContFilter  NVariant=InternalParameters  NCopyVariant=Disabled  FilterICVariant=InternalICsFilter  IntegratorICVariant=InternalICs  ExternalResetVariant=Disabled  TRSumVariant=Passthrough  SumFdbkVariant=Disabled  SumVariant=Sum_PID  TsampFilterVariant=InternalTs  TsampNgainVariant=Passthrough  TsampIntegralVariant=Disabled_SignalSpec  ExternalSaturationOutDataTypeStr=Inherit: Same as second input  DerivativeSourceVariant=ErrorSignal  PreIntVariant=InternalPreInt
  Saturation : Saturate  UpperLimit=57  LowerLimit=10 %-pump.negativeDisplacementLimit
  Sum : Sum  Inputs=|+-
  Target Velocity : Subsystem
  Transfer Fcn : TransferFcn  Denominator=[0.001 1]
  Pump Displacement : Outport
  wires:
  Tractor Vel/1 -> Transfer Fcn/1
  Transfer Fcn/1 -> Sum/2
  Saturation/1 -> Pump Displacement/1
  Sum/1 -> PID Controller/1
  PID Controller/1 -> Saturation/1
  Target Velocity/1(Target Vel) -> Sum/1

== system TractorTransmissionTradeOff/Driver Controls/Engine Speed Command ==
  Ramp : simulink/Sources/Ramp  slope=0.5*engine.speedRamp  start=0  InitialOutput=0
  Saturation1 : Saturate  UpperLimit=1.1*engine.upperLimit  LowerLimit=eps
  Engine Speed : Outport
  wires:
  Saturation1/1 -> Engine Speed/1
  Ramp/1 -> Saturation1/1

== system TractorTransmissionTradeOff/Driver Controls/Implement Depth Command ==
  Constant : Constant  Value=implement.depth3Tillage
  Depth Command : Outport
  wires:
  Constant/1 -> Depth Command/1

== system TractorTransmissionTradeOff/Implement/Terminators ==
  Inport : Inport
  Inport1 : Inport  Port=2
  Terminator : Terminator
  Terminator1 : Terminator
  wires:
  Inport/1 -> Terminator/1
  Inport1/1 -> Terminator1/1

== system TractorTransmissionTradeOff/Scenario/Front Left Tire Parameters ==
  note: tykc is tire-soil sinkage cohession moduli
      | tykphi is tire-soil sinkage friction moduli
      | tyn is tire-soil sinkage exponent
      | tc is soil cohesison coefficient
      | tk is soil shear deformation
      | tphi is soil internal shearling resistence angle
  Bus Creator : BusCreator  Inputs=tykc,tykphi,tyn,tc,tk,tphi
  tc : Constant  Value=tire.tc
  tk : Constant  Value=tire.tk
  tphi : Constant  Value=tire.tphi
  tykc : Constant  Value=tire.tykc
  tykphi : Constant  Value=tire.tykphi
  tyn : Constant  Value=tire.tyn
  Front Left Tire Bus : Outport
  wires:
  Bus Creator/1 -> Front Left Tire Bus/1
  tphi/1 -> Bus Creator/6  "tphi"
  tk/1 -> Bus Creator/5  "tk"
  tc/1 -> Bus Creator/4  "tc"
  tyn/1 -> Bus Creator/3  "tyn"
  tykphi/1 -> Bus Creator/2  "tykphi"
  tykc/1 -> Bus Creator/1  "tykc"

== system TractorTransmissionTradeOff/Scenario/Front Right Tire Parameters ==
  note: tykc is tire-soil sinkage cohession moduli
      | tykphi is tire-soil sinkage friction moduli
      | tyn is tire-soil sinkage exponent
      | tc is soil cohesison coefficient
      | tk is soil shear deformation
      | tphi is soil internal shearling resistence angle
  Bus Creator : BusCreator  Inputs=tykc,tykphi,tyn,tc,tk,tphi
  tc : Constant  Value=tire.tc
  tk : Constant  Value=tire.tk
  tphi : Constant  Value=tire.tphi
  tykc : Constant  Value=tire.tykc
  tykphi : Constant  Value=tire.tykphi
  tyn : Constant  Value=tire.tyn
  Front Right Tire Bus : Outport
  wires:
  tykc/1 -> Bus Creator/1  "tykc"
  tykphi/1 -> Bus Creator/2  "tykphi"
  tyn/1 -> Bus Creator/3  "tyn"
  tc/1 -> Bus Creator/4  "tc"
  tk/1 -> Bus Creator/5  "tk"
  tphi/1 -> Bus Creator/6  "tphi"
  Bus Creator/1 -> Front Right Tire Bus/1

== system TractorTransmissionTradeOff/Scenario/Implement-Soil Scenario ==
  Constant : Constant  Value=textureID
  Implement-Soil Parameter : Outport
  wires:
  Constant/1 -> Implement-Soil Parameter/1  "soil_texture"

== system TractorTransmissionTradeOff/Scenario/Rear Right Tire Parameters ==
  note: tykc is tire-soil sinkage cohession moduli
      | tykphi is tire-soil sinkage friction moduli
      | tyn is tire-soil sinkage exponent
      | tc is soil cohesison coefficient
      | tk is soil shear deformation
      | tphi is soil internal shearling resistence angle
  Bus Creator : BusCreator  Inputs=tykc,tykphi,tyn,tc,tk,tphi
  tc : Constant  Value=tire.tc
  tk : Constant  Value=tire.tk
  tphi : Constant  Value=tire.tphi
  tykc : Constant  Value=tire.tykc
  tykphi : Constant  Value=tire.tykphi
  tyn : Constant  Value=tire.tyn
  Rear Right Tire Bus : Outport
  wires:
  Bus Creator/1 -> Rear Right Tire Bus/1
  tphi/1 -> Bus Creator/6  "tphi"
  tk/1 -> Bus Creator/5  "tk"
  tc/1 -> Bus Creator/4  "tc"
  tyn/1 -> Bus Creator/3  "tyn"
  tykphi/1 -> Bus Creator/2  "tykphi"
  tykc/1 -> Bus Creator/1  "tykc"

== system TractorTransmissionTradeOff/Scenario/RearLeft Tire Parameters ==
  note: tykc is tire-soil sinkage cohession moduli
      | tykphi is tire-soil sinkage friction moduli
      | tyn is tire-soil sinkage exponent
      | tc is soil cohesison coefficient
      | tk is soil shear deformation
      | tphi is soil internal shearling resistence angle
  Bus Creator : BusCreator  Inputs=tykc,tykphi,tyn,tc,tk,tphi
  tc : Constant  Value=tire.tc
  tk : Constant  Value=tire.tk
  tphi : Constant  Value=tire.tphi
  tykc : Constant  Value=tire.tykc
  tykphi : Constant  Value=tire.tykphi
  tyn : Constant  Value=tire.tyn
  Rear Left Tire Bus : Outport
  wires:
  tykc/1 -> Bus Creator/1  "tykc"
  tykphi/1 -> Bus Creator/2  "tykphi"
  tyn/1 -> Bus Creator/3  "tyn"
  tphi/1 -> Bus Creator/6  "tphi"
  Bus Creator/1 -> Rear Left Tire Bus/1
  tc/1 -> Bus Creator/4  "tc"
  tk/1 -> Bus Creator/5  "tk"

== system TractorTransmissionTradeOff/Scenario/Road Inclination Scenario ==
  Ramp : simulink/Sources/Ramp  slope=2*pi/180/15  start=0  InitialOutput=0
  Ramp1 : simulink/Sources/Ramp  slope=-2*pi/180/15  start=105  InitialOutput=0
  Saturation : Saturate  UpperLimit=2*pi/180  LowerLimit=0
  Saturation1 : Saturate  UpperLimit=0  LowerLimit=-2*pi/180
  Sum : Sum  Inputs=|++
  Transfer Fcn : TransferFcn  Denominator=[1 1]
  Scenario : Outport
  wires:
  Sum/1 -> Transfer Fcn/1
  Transfer Fcn/1 -> Scenario/1
  Ramp/1 -> Saturation/1
  Ramp1/1 -> Saturation1/1
  Saturation/1 -> Sum/1
  Saturation1/1 -> Sum/2

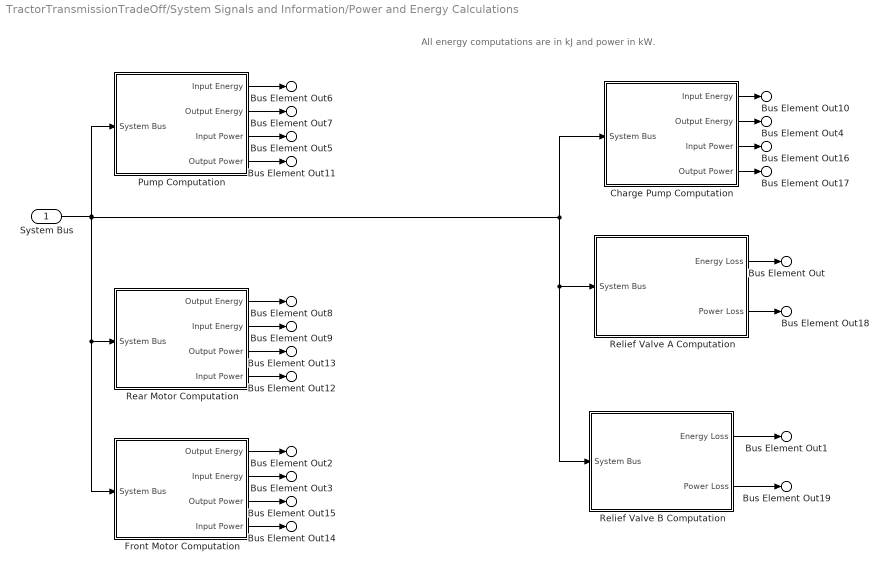
== system TractorTransmissionTradeOff/System Signals and Information/Power and Energy Calculations ==
  note: All energy computations are in kJ and power in kW.
  System Bus : Inport
  Charge Pump Computation : Subsystem
  Front Motor Computation : Subsystem
  Pump Computation : Subsystem
  Rear Motor Computation : Subsystem
  Relief Valve A Computation : Subsystem
  Relief Valve B Computation : Subsystem
  Bus Element Out : Outport  PortName=Energy Bus  Element=Energy Loss Relief A
  Bus Element Out1 : Outport  PortName=Energy Bus  Element=Energy Loss Relief B
  Bus Element Out6 : Outport  PortName=Energy Bus  Element=Pump Total Input Energy
  Bus Element Out7 : Outport  PortName=Energy Bus  Element=Pump Total Output Energy
  Bus Element Out8 : Outport  PortName=Energy Bus  Element=Rear Motor Total Output Energy
  Bus Element Out9 : Outport  PortName=Energy Bus  Element=Rear Motor Total Input Energy
  Bus Element Out2 : Outport  PortName=Energy Bus  Element=Front Motor Total Output Energy
  Bus Element Out3 : Outport  PortName=Energy Bus  Element=Front Motor Total Input Energy
  Bus Element Out10 : Outport  PortName=Energy Bus  Element=Charge Pump Input Energy
  Bus Element Out4 : Outport  PortName=Energy Bus  Element=Charge Pump Output Energy
  Bus Element Out5 : Outport  Port=2  PortName=Power Bus  Element=Pump Total Input Power
  Bus Element Out11 : Outport  Port=2  PortName=Power Bus  Element=Pump Total Output Power
  Bus Element Out12 : Outport  Port=2  PortName=Power Bus  Element=Rear Motor Total Input Power
  Bus Element Out13 : Outport  Port=2  PortName=Power Bus  Element=Rear Motor Total Output Power
  Bus Element Out14 : Outport  Port=2  PortName=Power Bus  Element=Front Motor Total Input Power
  Bus Element Out15 : Outport  Port=2  PortName=Power Bus  Element=Front Motor Total Output Power
  Bus Element Out16 : Outport  Port=2  PortName=Power Bus  Element=Charge Pump Total Input Power
  Bus Element Out17 : Outport  Port=2  PortName=Power Bus  Element=Charge Pump Total Output Power
  Bus Element Out18 : Outport  Port=2  PortName=Power Bus  Element=Power Loss Relief A
  Bus Element Out19 : Outport  Port=2  PortName=Power Bus  Element=Power Loss Relief B
  wires:
  System Bus/1 -> Front Motor Computation/1(System Bus), Rear Motor Computation/1(System Bus), Charge Pump Computation/1(System Bus), Relief Valve B Computation/1(System Bus), Relief Valve A Computation/1(System Bus), Pump Computation/1(System Bus)
  Relief Valve A Computation/1("Energy Loss ") -> Bus Element Out/1
  Relief Valve B Computation/1("Energy Loss ") -> Bus Element Out1/1
  Pump Computation/1(Input Energy) -> Bus Element Out6/1
  Pump Computation/2("Output Energy ") -> Bus Element Out7/1
  Rear Motor Computation/1(Output Energy) -> Bus Element Out8/1
  Rear Motor Computation/2("Input Energy  ") -> Bus Element Out9/1
  Front Motor Computation/1(Output Energy) -> Bus Element Out2/1
  Front Motor Computation/2("Input Energy ") -> Bus Element Out3/1
  Charge Pump Computation/1(Input Energy) -> Bus Element Out10/1
  Charge Pump Computation/2("Output Energy ") -> Bus Element Out4/1
  Pump Computation/3(Input Power) -> Bus Element Out5/1
  Pump Computation/4(Output Power) -> Bus Element Out11/1
  Rear Motor Computation/4(Input Power) -> Bus Element Out12/1
  Rear Motor Computation/3(Output Power) -> Bus Element Out13/1
  Front Motor Computation/3(Output Power) -> Bus Element Out15/1
  Front Motor Computation/4(Input Power) -> Bus Element Out14/1
  Charge Pump Computation/4(Output Power) -> Bus Element Out17/1
  Charge Pump Computation/3(Input Power) -> Bus Element Out16/1
  Relief Valve A Computation/2(Power Loss) -> Bus Element Out18/1
  Relief Valve B Computation/2("Power Loss ") -> Bus Element Out19/1

== system TractorTransmissionTradeOff/Tractor/Front Axle ==
  Front Differential : sdl_lib/Gears/Differential  driveshaft_location=sdl.enum.differential_orientation.right  cd_ratio=finalDrive.gearRatioFront  friction_model=sdl.enum.gear_friction.none  efficiency=[ 0.85 0.92 ]  temperature_TLU=[ 280 300 320 ] K  efficiency_ss_TLU=[ 0.95 0.9 0.85 ]  efficiency_cd_TLU=[ 0.95 0.9 0.85 ]  pwr_thr=[ 0.001 0.001 ] W  mu_visc=[ 0 0 ] N*m/(rad/s)  model_inertia=simscape.enum.onoff.on  sun_inertia=1e-10 kg*m^2  sun_radius=0.01 m  carrier_inertia=0.1 kg*m^2  planet_inertia=0.1 kg*m^2  planet_mass=1e-10 kg  thermal_mass=50 J/K  T_init=300 K
  "  " : PMIOPort  Side=Left
  AF : PMIOPort  Port=2  Side=Right
  " " : PMIOPort  Port=3  Side=Right
  connections:
  Front Differential/RConn1 -- "  "/RConn1
  Front Differential/RConn2 -- " "/RConn1
  AF/RConn1 -- Front Differential/LConn1

== system TractorTransmissionTradeOff/Tractor/Rear Axle ==
  Rear Differential : sdl_lib/Gears/Differential  driveshaft_location=sdl.enum.differential_orientation.right  cd_ratio=finalDrive.gearRatioRear  friction_model=sdl.enum.gear_friction.none  efficiency=[ 0.85 0.92 ]  temperature_TLU=[ 280 300 320 ] K  efficiency_ss_TLU=[ 0.95 0.9 0.85 ]  efficiency_cd_TLU=[ 0.95 0.9 0.85 ]  pwr_thr=[ 0.001 0.001 ] W  mu_visc=[ 0 0 ] N*m/(rad/s)  model_inertia=simscape.enum.onoff.on  sun_inertia=1e-10 kg*m^2  sun_radius=0.01 m  carrier_inertia=0.1 kg*m^2  planet_inertia=0.1 kg*m^2  planet_mass=1e-10 kg  thermal_mass=50 J/K  T_init=300 K
  " " : PMIOPort  Side=Left
  AR : PMIOPort  Port=2  Side=Right
  "  " : PMIOPort  Port=3  Side=Right
  connections:
  "  "/RConn1 -- Rear Differential/RConn2
  Rear Differential/RConn1 -- " "/RConn1
  AR/RConn1 -- Rear Differential/LConn1

== system TractorTransmissionTradeOff/Tractor/Tire FL ==
  S : Inport
  Bus Selector : BusSelector  OutputSignals=Front Left Tire.tc,Front Left Tire.tphi,Front Left Tire.tk,Front Left Tire.tyn,Front Left Tire.tykphi,Front Left Tire.tykc
  Simulink-PS Converter : nesl_utility/Simulink-PS Converter  PhysicalDomain=network_engine_domain  SubClassName=ps_input  LeftPortType=input  RightPortType=output  PseudoPeriodic=off  Frequencies=[]  NoiseDistribution=none  NoiseParameters=[]  Unit=kN/m^2  AffineConversion=off  FilteringAndDerivatives=provide  SimscapeFilterOrder=1  InputFilterTimeConstant=0.001  UdotUserProvided=0
  Simulink-PS Converter1 : nesl_utility/Simulink-PS Converter  PhysicalDomain=network_engine_domain  SubClassName=ps_input  LeftPortType=input  RightPortType=output  PseudoPeriodic=off  Frequencies=[]  NoiseDistribution=none  NoiseParameters=[]  Unit=deg  AffineConversion=off  FilteringAndDerivatives=provide  SimscapeFilterOrder=1  InputFilterTimeConstant=0.001  UdotUserProvided=0
  Simulink-PS Converter2 : nesl_utility/Simulink-PS Converter  PhysicalDomain=network_engine_domain  SubClassName=ps_input  LeftPortType=input  RightPortType=output  PseudoPeriodic=off  Frequencies=[]  NoiseDistribution=none  NoiseParameters=[]  Unit=cm  AffineConversion=off  FilteringAndDerivatives=provide  SimscapeFilterOrder=1  InputFilterTimeConstant=0.001  UdotUserProvided=0
  Simulink-PS Converter3 : nesl_utility/Simulink-PS Converter  PhysicalDomain=network_engine_domain  SubClassName=ps_input  LeftPortType=input  RightPortType=output  PseudoPeriodic=off  Frequencies=[]  NoiseDistribution=none  NoiseParameters=[]  Unit=1  AffineConversion=off  FilteringAndDerivatives=provide  SimscapeFilterOrder=1  InputFilterTimeConstant=0.001  UdotUserProvided=0
  Simulink-PS Converter4 : nesl_utility/Simulink-PS Converter  PhysicalDomain=network_engine_domain  SubClassName=ps_input  LeftPortType=input  RightPortType=output  PseudoPeriodic=off  Frequencies=[]  NoiseDistribution=none  NoiseParameters=[]  Unit=1  AffineConversion=off  FilteringAndDerivatives=provide  SimscapeFilterOrder=1  InputFilterTimeConstant=0.001  UdotUserProvided=0
  Simulink-PS Converter5 : nesl_utility/Simulink-PS Converter  PhysicalDomain=network_engine_domain  SubClassName=ps_input  LeftPortType=input  RightPortType=output  PseudoPeriodic=off  Frequencies=[]  NoiseDistribution=none  NoiseParameters=[]  Unit=1  AffineConversion=off  FilteringAndDerivatives=provide  SimscapeFilterOrder=1  InputFilterTimeConstant=0.001  UdotUserProvided=0
  Tire FL : SimscapeComponentBlock  SourceFile=tire_soil  ComponentPath=tire_soil  ComponentVariants="[\"tire_soil\"]"  ComponentVariantNames="[\"tire_soil\"]"  ClassName=tire_soil  SchemaVersion=1  load_TLU="tire.loadVector  kN"  p_inflation_TLU=tire.inflationPressureVector kPa  deflection_TLU="tire.deflectionTable  cm"  area_TLU="tire.contactPatchArea  cm^2"  inflation_pressure=tire.inflationPressure kPa  k_e=tire.constructionCoefficient  r_e=tire.rollingRadiusFront m  bti=tire.sectionWidth m  hti=tire.sectionHeight m  model_compliance=sdl.enum.compliance.off  stiffness=1e6 N/m  damping=1000 N*s/m  model_inertia=sdl.enum.model_inertia.off  inertia=2 kg*m^2  initial_velocity=0 rad/s  vxlow=1 m/s  v_tr_thr=0.001 m/s  kpumin=-1.5  kpumax=1.5  p_thr=0.01 bar  b_thr=1 mm  r_e_t=0.5 m  rolling_radius_model=sdl.enum.RollingRadiusParameterization.Constant  fz0=4000 N  r_0=0.5 m  breff=8.39  dreff=0.26  freff=0.074  q_re0=0.99  q_v1=0.008  longvl=17 m/s  cz=5e5 N/m
      settings: CopyFcn=simscape.sscblock.internal.componentBlockCallback(gcbh,'COPY')  PreCopyFcn=simscape.sscblock.internal.componentBlockCallback(gcbh,'PRECOPY')  PreDeleteFcn=simscape.sscblock.internal.componentBlockCallback(gcbh,'PREDELETE')  InternalSimscapePortConfiguration="{\"Bottom\":[{\"id\":\"tykc\",\"label\":\"tykc\",\"type\":\"input\"},{\"id\":\"tykphi\",\"label\":\"tykphi\",\"type\":\"input\"},{\"id\":\"tyn\",\"label\":\"tyn\",\"type\":\"input\"}],\"Left\":[{\"id\":\"A\",\"label\":\"A\",\"type\":\"foundation.mechanical.rotational.rotational\"},{\"id\":\"H\",\"label\":\"H\",\"type\":\"foundation.mechanical.translational.translational\"}],\"Right\":[{\"id\":\"S\",\"label\":\"S\",\"type\":\"output\"}],\"Top\":[{\"id\":\"N\",\"label\":\"N\",\"type\":\"input\"},{\"id\":\"tc\",\"label\":\"tc\",\"type\":\"input\"},{\"id\":\"tphi\",\"label\":\"tphi\",\"type\":\"input\"},{\"id\":\"tk\",\"label\":\"tk\",\"type\":\"input\"}]}"
      mask Type: Tire (Tire-Soil)
  H : PMIOPort  Side=Left
  N : PMIOPort  Port=2  Side=Left
  FLT : PMIOPort  Port=3  Side=Right
  wires:
  S/1 -> Bus Selector/1
  Bus Selector/1 -> Simulink-PS Converter/1  "<tc>"
  Bus Selector/2 -> Simulink-PS Converter1/1  "<tphi>"
  Bus Selector/3 -> Simulink-PS Converter2/1  "<tk>"
  Bus Selector/4 -> Simulink-PS Converter3/1  "<tyn>"
  Bus Selector/5 -> Simulink-PS Converter4/1  "<tykphi>"
  Bus Selector/6 -> Simulink-PS Converter5/1  "<tykc>"
  connections:
  Simulink-PS Converter/RConn1 -- Tire FL/LConn4
  Simulink-PS Converter1/RConn1 -- Tire FL/LConn5
  Simulink-PS Converter2/RConn1 -- Tire FL/LConn6
  Simulink-PS Converter3/RConn1 -- Tire FL/RConn4
  Simulink-PS Converter4/RConn1 -- Tire FL/RConn3
  Simulink-PS Converter5/RConn1 -- Tire FL/RConn2
  N/RConn1 -- Tire FL/LConn3
  FLT/RConn1 -- Tire FL/LConn1
  H/RConn1 -- Tire FL/LConn2
